simulink model "ElectroMechanics_Q_modified"  (R2024a)
settings: Solver=VariableStepAuto  StartTime=0.0  StopTime=40  RelTol=1e-3
libraries: fl_lib x15, nesl_utility x11, sdl_lib x4, ee_lib x4, batteryecm_lib x1, simulink x1
(part 2 of 2)

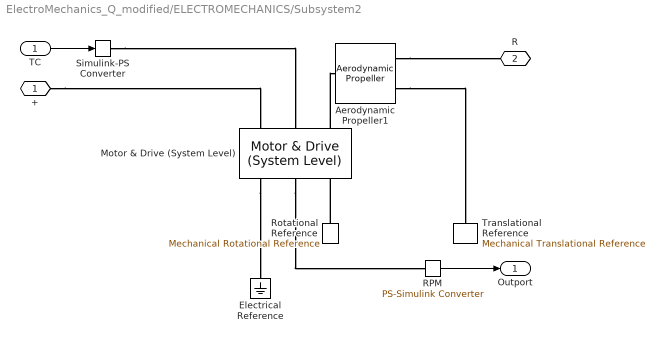
== system ElectroMechanics_Q_modified/ELECTROMECHANICS/Subsystem2 ==
  TC : Inport
  " Electrical Reference" : fl_lib/Electrical/Electrical Elements/Electrical Reference
  Aerodynamic Propeller1 : sdl_lib/Engines & Motors/Aerodynamic Propeller  parameterization=sdl.enum.AerodynamicPropellerParameterization.Constant  pitch_type=foundation.enum.constant_controlled.constant  direction=sdl.enum.PropellerDirection.Positive  root_pitch=0 deg  D=0.254 m  kt_const=0.110  kp_const=0.05655  kt_poly_fixed=[.002, .0006, -.0509, .0617]  kp_poly_fixed=[-.0752, .0577, -.0622, .16]  pitch_angle_TLU=[-15, 15, 25, 35, 45] deg  kt_poly_TLU=[.0002, -.00041, -.036, .03; .00026, -.00056, -.048, .04; .002, .00063, -.051, .062; .0014, -.0016, -.048, .087; .00087, -.0036, -.041, .12]  kp_poly_TLU=[-.1, .031, .0055, .088; -.081, -.025, .0044, .07; -.075, .058, -.062, .16; -.052, .065, -.08, .3; -.031, .057, -.069, .4]  J_TLU=[.01, .3, .625, 1.55, 2, 2.6]  kt_TLU_1D=[.0614, .0473, .0318, -.0127, -.0343, -.063]  kp_TLU_1D=[.1496, .1314, .116, -.0521, -.1503, -.2813]  kt_TLU_2D=[.00019, .013, .0048, -.017, -.03, -.045; .00039, .025, .0096, -.037, -.06, -.09; .00061, .047, .032, -.013, -.034, -.063; .00086, .072, .057, .014, -.0076, -.036; .12, .104, .09, .049, .029, .0019]  kp_TLU_2D=[.029, .029, .016, .06, .009, -.16; .059, .054, .031, -.12, -.19, -.29; .15, .13, .12, -.052, -.15, -.28; .26, .24, .22, .097, -.04, -.25; .39, .39, .38, .32, .24, .062]  beta_TLU=linspace(0, 360, 10) deg  Ct_TLU_1D=0.035 * sind(linspace(0, 360, 10) - 200)  Cq_TLU_1D=0.010 * sind(linspace(0, 360, 10) - 200)  Ct_TLU_2D=[0.01 * sind(linspace(0, 360, 10) - 200); 0.020 * sind(linspace(0, 360, 10) - 200); 0.035 * sind(linspace(0, 360, 10) - 200); 0.04 * sind(linspace(0, 360, 10) - 200); 0.06 * sind(linspace(0, 360, 10) - 200)]  Cq_TLU_2D=[0.0005 * sind(linspace(0, 360, 10) - 200); 0.0015 * sind(linspace(0, 360, 10) - 200); 0.0025 * sind(linspace(0, 360, 10) - 200); 0.0035 * sind(linspace(0, 360, 10) - 200); 0.0045 * sind(linspace(0, 360, 10) - 200)]  n_blades=2  n_blade_discretization=20  radial_TLU=[.1, .12, .2, .4, .6, .8, 1]  twist_TLU=[30, 35, 50, 30, 20, 15, 10] deg  chord_TLU=[.0676, .0666, .0824, .1025, .0885, .0598, .0133]  alpha_TLU=-180 : 10 : 180 deg  Cl_TLU=[.1326, .1326, .1274, .1274, .1274, .1274, .1274; .3626, .3626, .5002, .5002, .5002, .5002, .5002; .5528, .5528, .8007, .8007, .8007, .8007, .8007; .7256, .7256, 1.0125, 1.0125, 1.0125, 1.0125, 1.0125; .8016, .8016, 1.1556, 1.1556, 1.1556, 1.1556, 1.1556; .7873, .7873, 1.1604, 1.1604, 1.1604, 1.1604, 1.1604; .7031, .7031, 1.0493, 1.0493, 1.0493, 1.0493, 1.0493; .5423, .5423, .7973, .7973, .7973, .7973, .7973; .3537, .3537, .4332, .4332, .4332, .4332, .4332; .1155, .1155, -.0376, -.0376, -.0376, -.0376, -.0376; -.1045, -.1045, -.4096, -.4096, -.4096, -.4096, -.4096; -.2999, -.2999, -.672, -.672, -.672, -.672, -.672; -.4401, -.4401, -.9343, -.9343, -.9343, -.9343, -.9343; -.5186, -.5186, -1.0477, -1.0477, -1.0477, -1.0477, -1.0477; -.5303, -.5303, -1.0387, -1.0387, -1.0387, -1.0387, -1.0387; -.5073, -.5073, -.9565, -.9565, -.9565, -.9565, -.9565; -.442, -.442, -.7713, -.7713, -.7713, -.7713, -.7713; -.2658, -.2658, -.4832, -.4832, -.4832, -.4832, -.4832; .4109, .4109, .3629, .3629, .3629, .3629, .3629; 1.1635, 1.1635, 1.3779, 1.3779, 1.3779, 1.3779, 1.3779; 1.2412, 1.2412, 1.4033, 1.4033, 1.4033, 1.4033, 1.4033; .7434, .7434, 1.3453, 1.3453, 1.3453, 1.3453, 1.3453; .7908, .7908, 1.2862, 1.2862, 1.2862, 1.2862, 1.2862; .7525, .7525, 1.1562, 1.1562, 1.1562, 1.1562, 1.1562; .6722, .6722, .9487, .9487, .9487, .9487, .9487; .5324, .5324, .7047, .7047, .7047, .7047, .7047; .3365, .3365, .382, .382, .382, .382, .382; .0529, .0529, -.0229, -.0229, -.0229, -.0229, -.0229; -.2728, -.2728, -.316, -.316, -.316, -.316, -.316; -.4135, -.4135, -.6195, -.6195, -.6195, -.6195, -.6195; -.5087, -.5087, -.7847, -.7847, -.7847, -.7847, -.7847; -.5342, -.5342, -.8419, -.8419, -.8419, -.8419, -.8419; -.5166, -.5166, -.7658, -.7658, -.7658, -.7658, -.7658; -.4321, -.4321, -.5707, -.5707, -.5707, -.5707, -.5707; -.2864, -.2864, -.3098, -.3098, -.3098, -.3098, -.3098; -.1073, -.1073, -.0893, -.0893, -.0893, -.0893, -.0893; .1326, .1326, .1274, .1274, .1274, .1274, .1274]  Cd_TLU=[.0055, .0055, .3904, .3904, .3904, .3904, .3904; .0774, .0774, .449, .449, .449, .449, .449; .2412, .2412, .5915, .5915, .5915, .5915, .5915; .4342, .4342, .8307, .8307, .8307, .8307, .8307; .679, .679, 1.0909, 1.0909, 1.0909, 1.0909, 1.0909; .9003, .9003, 1.3868, 1.3868, 1.3868, 1.3868, 1.3868; 1.0825, 1.0825, 1.6565, 1.6565, 1.6565, 1.6565, 1.6565; 1.2281, 1.2281, 1.875, 1.875, 1.875, 1.875, 1.875; 1.3205, 1.3205, 2.017, 2.017, 2.017, 2.017, 2.017; 1.3234, 1.3234, 2.0407, 2.0407, 2.0407, 2.0407, 2.0407; 1.2391, 1.2391, 1.9513, 1.9513, 1.9513, 1.9513, 1.9513; 1.0963, 1.0963, 1.7643, 1.7643, 1.7643, 1.7643, 1.7643; .8978, .8978, 1.5048, 1.5048, 1.5048, 1.5048, 1.5048; .6525, .6525, 1.2281, 1.2281, 1.2281, 1.2281, 1.2281; .4203, .4203, .838, .838, .838, .838, .838; .2428, .2428, .5434, .5434, .5434, .5434, .5434; .0951, .0951, .2517, .2517, .2517, .2517, .2517; .0292, .0292, .0698, .0698, .0698, .0698, .0698; .0148, .0148, .0267, .0267, .0267, .0267, .0267; .0808, .0808, .0509, .0509, .0509, .0509, .0509; .2429, .2429, .1561, .1561, .1561, .1561, .1561; .5019, .5019, .3927, .3927, .3927, .3927, .3927; .7217, .7217, .7438, .7438, .7438, .7438, .7438; .9336, .9336, 1.1277, 1.1277, 1.1277, 1.1277, 1.1277; 1.0984, 1.0984, 1.4838, 1.4838, 1.4838, 1.4838, 1.4838; 1.2274, 1.2274, 1.7877, 1.7877, 1.7877, 1.7877, 1.7877; 1.3016, 1.3016, 1.9779, 1.9779, 1.9779, 1.9779, 1.9779; 1.3305, 1.3305, 2.0516, 2.0516, 2.0516, 2.0516, 2.0516; 1.2889, 1.2889, 1.9974, 1.9974, 1.9974, 1.9974, 1.9974; 1.1677, 1.1677, 1.8463, 1.8463, 1.8463, 1.8463, 1.8463; 1.0076, 1.0076, 1.5699, 1.5699, 1.5699, 1.5699, 1.5699; .8068, .8068, 1.2596, 1.2596, 1.2596, 1.2596, 1.2596; .5688, .5688, .9493, .9493, .9493, .9493, .9493; .3604, .3604, .6154, .6154, .6154, .6154, .6154; .1802, .1802, .5015, .5015, .5015, .5015, .5015; .0699, .0699, .4265, .4265, .4265, .4265, .4265; .0055, .0055, .3904, .3904, .3904, .3904, .3904]  interp_method=simscape.enum.interpolation.linear  extrap_method=simscape.enum.extrapolation.linear  density_spec=foundation.enum.constant_variable.constant  rho=1.225 kg/m^3  rotational_ports=sdl.enum.ConnectionType.Conserving  translational_ports=sdl.enum.ConnectionType.Conserving  model_inertia=true  propeller_inertia=0.00005 kg*m^2  propeller_mass=15 g  efficiency_sensor=false  n_thr=0.001 Hz  k_thr=0.001  P_thr=0.01 W  operation_check=simscape.enum.assert.action.warn  expose_port_C=false  w_specify=off  w_priority=None  w=0 rad/s  w_nominal_specify=off  w_nominal_value=1  w_nominal_unit=rad/s  Q_specify=off  Q_priority=None  Q=0 N*m  Q_nominal_specify=off  Q_nominal_value=1  Q_nominal_unit=N*m  v_specify=off  v_priority=None  v=0 m/s  v_nominal_specify=off  v_nominal_value=1  v_nominal_unit=m/s  thrust_specify=off  thrust_priority=None  thrust=0 N  thrust_nominal_specify=off  thrust_nominal_value=1  thrust_nominal_unit=N
      settings: InternalSimscapePortConfiguration="{\"Bottom\":[],\"Left\":[{\"id\":\"R1\",\"label\":\"R1\",\"type\":\"foundation.mechanical.rotational.rotational\"}],\"Right\":[{\"id\":\"R2\",\"label\":\"R2\",\"type\":\"foundation.mechanical.translational.translational\"},{\"id\":\"C2\",\"label\":\"C2\",\"type\":\"foundation.mechanical.translational.translational\"}],\"Top\":[]}"
  Motor & Drive (System Level) : ee_lib/Electromechanical/Motor & Drive (System Level)  torque_speed_param=ee.enum.electromech.envelope.torque_power  overtorque_param=ee.enum.electromech.overtorque.no  T_t=[.09, .08, .07, 0] N*m  T_t_intermittent=[.36, .32, .28, 0] N*m  T_t_2D=[.09, .09, .09; .08, .08, .08; .07, .07, .07; 0, 0, 0] N*m  T_t_intermittent_2D=[.36, .36, .36; .32, .32, .32; .28, .28, .28; 0, 0, 0] N*m  w_t=[0, 3750, 7500, 8000] rpm  vdc_t=[6, 12, 24] V  torque_max=0.5 N*m  power_max=450 W  torque_max_intermittent=0.4 N*m  power_max_intermittent=120 W  time_overtorque=30 s  time_recover=60 s  Tc=0.005 s  EnableSwitch=false  losses_param=1  eff=95  w_eff=6000 rpm  T_eff=116.5 mN*m  Piron=0 W  Pbase=0 W  w_eff_vec=[-8000, -4000, 0, 4000, 8000] rpm  T_eff_vec=[0, .03, .06, .09] N*m  v_eff_vec=[100, 250, 400] V  losses_mat=[1.49, 1.67, 2.21, 3.1; .42, .69, 1.14, 2.03; .06, .24, .78, 1.68; .42, .69, 1.14, 2.03; 1.49, 1.67, 2.21, 3.1] W  efficiency_mat=[95, 95, 95, 95; 95, 95, 95, 95; 95, 95, 95, 95; 95, 95, 95, 95; 95, 95, 95, 95]  losses_mat_3D=ones(5, 4, 3) W  efficiency_mat_3D=95 * ones(5, 4, 3)  Res=0.085 Ohm  enable_fault=simscape.enum.onoff.off  fault_condition=1  fault_threshold=0.5  J=1.5e-5 kg*m^2  lam=2.5e-8 N*m*s/rad  speed0=0 rpm  faulted_specify=off  faulted_priority=None  faulted=0  faulted_nominal_specify=off  faulted_nominal_value=1  faulted_nominal_unit=1  isSwitchedOff_specify=off  isSwitchedOff_priority=None  isSwitchedOff=0  isSwitchedOff_nominal_specify=off  isSwitchedOff_nominal_value=1  isSwitchedOff_nominal_unit=1  torqueLimitContinuous_specify=off  torqueLimitContinuous_priority=None  torqueLimitContinuous=0 N*m  torqueLimitContinuous_nominal_specify=off  torqueLimitContinuous_nominal_value=1  torqueLimitContinuous_nominal_unit=N*m  alpha=3.93e-3 1/K  Tmeas=25 degC  Tmeas2=125 degC  losses_mat_T2=[1.49, 1.74, 2.49, 3.74; .42, .67, 1.42, 2.67; .06, .31, 1.06, 2.31; .42, .67, 1.42, 2.67; 1.49, 1.74, 2.49, 3.74] W  efficiency_mat_T2=[95, 95, 95, 95; 95, 95, 95, 95; 95, 95, 95, 95; 95, 95, 95, 95; 95, 95, 95, 95]  losses_mat_3D_T2=ones(5, 4, 3) W  efficiency_mat_3D_T2=95 * ones(5, 4, 3)  thermal_mass=100 J/K  initial_temperature=25 degC
  RPM : nesl_utility/PS-Simulink Converter  PhysicalDomain=network_engine_domain  SubClassName=ps_output  LeftPortType=input  RightPortType=output  PseudoPeriodic=off  Frequencies=[]  VectorFormat=inherit  Unit=rpm  AffineConversion=off
  Rotational Reference : fl_lib/Mechanical/Rotational Elements/Mechanical Rotational Reference
  Simulink-PS Converter : nesl_utility/Simulink-PS Converter  PhysicalDomain=network_engine_domain  SubClassName=ps_input  LeftPortType=input  RightPortType=output  PseudoPeriodic=off  Frequencies=[]  NoiseDistribution=none  NoiseParameters=[]  Unit=1  AffineConversion=off  FilteringAndDerivatives=provide  SimscapeFilterOrder=1  InputFilterTimeConstant=0.001  UdotUserProvided=0
  Translational Reference : fl_lib/Mechanical/Translational Elements/Mechanical Translational Reference
  + : PMIOPort  Side=Left
  R : PMIOPort  Port=2  Side=Right
  Outport : Outport
  wires:
  RPM/1 -> Outport/1
  TC/1 -> Simulink-PS Converter/1
  connections:
  Aerodynamic Propeller1/RConn2 -- Translational Reference/LConn1
  Rotational Reference/LConn1 -- Motor & Drive (System Level)/RConn3
  Motor & Drive (System Level)/RConn1 -- " Electrical Reference"/LConn1
  Motor & Drive (System Level)/LConn3 -- Aerodynamic Propeller1/LConn1
  Motor & Drive (System Level)/RConn2 -- RPM/LConn1
  +/RConn1 -- Motor & Drive (System Level)/LConn1
  Aerodynamic Propeller1/RConn1 -- R/RConn1
  Simulink-PS Converter/RConn1 -- Motor & Drive (System Level)/LConn2

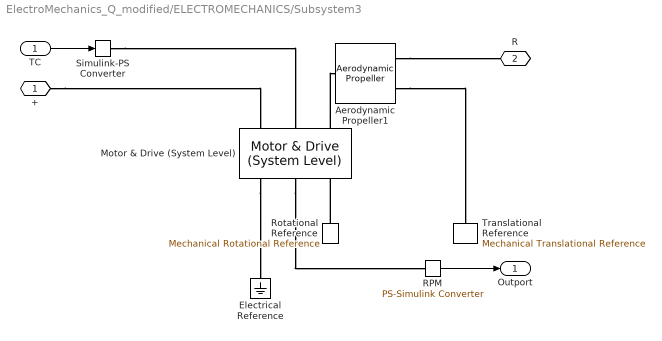
== system ElectroMechanics_Q_modified/ELECTROMECHANICS/Subsystem3 ==
  TC : Inport
  " Electrical Reference" : fl_lib/Electrical/Electrical Elements/Electrical Reference
  Aerodynamic Propeller1 : sdl_lib/Engines & Motors/Aerodynamic Propeller  parameterization=sdl.enum.AerodynamicPropellerParameterization.Constant  pitch_type=foundation.enum.constant_controlled.constant  direction=sdl.enum.PropellerDirection.Positive  root_pitch=0 deg  D=0.254 m  kt_const=0.110  kp_const=0.05655  kt_poly_fixed=[.002, .0006, -.0509, .0617]  kp_poly_fixed=[-.0752, .0577, -.0622, .16]  pitch_angle_TLU=[-15, 15, 25, 35, 45] deg  kt_poly_TLU=[.0002, -.00041, -.036, .03; .00026, -.00056, -.048, .04; .002, .00063, -.051, .062; .0014, -.0016, -.048, .087; .00087, -.0036, -.041, .12]  kp_poly_TLU=[-.1, .031, .0055, .088; -.081, -.025, .0044, .07; -.075, .058, -.062, .16; -.052, .065, -.08, .3; -.031, .057, -.069, .4]  J_TLU=[.01, .3, .625, 1.55, 2, 2.6]  kt_TLU_1D=[.0614, .0473, .0318, -.0127, -.0343, -.063]  kp_TLU_1D=[.1496, .1314, .116, -.0521, -.1503, -.2813]  kt_TLU_2D=[.00019, .013, .0048, -.017, -.03, -.045; .00039, .025, .0096, -.037, -.06, -.09; .00061, .047, .032, -.013, -.034, -.063; .00086, .072, .057, .014, -.0076, -.036; .12, .104, .09, .049, .029, .0019]  kp_TLU_2D=[.029, .029, .016, .06, .009, -.16; .059, .054, .031, -.12, -.19, -.29; .15, .13, .12, -.052, -.15, -.28; .26, .24, .22, .097, -.04, -.25; .39, .39, .38, .32, .24, .062]  beta_TLU=linspace(0, 360, 10) deg  Ct_TLU_1D=0.035 * sind(linspace(0, 360, 10) - 200)  Cq_TLU_1D=0.010 * sind(linspace(0, 360, 10) - 200)  Ct_TLU_2D=[0.01 * sind(linspace(0, 360, 10) - 200); 0.020 * sind(linspace(0, 360, 10) - 200); 0.035 * sind(linspace(0, 360, 10) - 200); 0.04 * sind(linspace(0, 360, 10) - 200); 0.06 * sind(linspace(0, 360, 10) - 200)]  Cq_TLU_2D=[0.0005 * sind(linspace(0, 360, 10) - 200); 0.0015 * sind(linspace(0, 360, 10) - 200); 0.0025 * sind(linspace(0, 360, 10) - 200); 0.0035 * sind(linspace(0, 360, 10) - 200); 0.0045 * sind(linspace(0, 360, 10) - 200)]  n_blades=2  n_blade_discretization=20  radial_TLU=[.1, .12, .2, .4, .6, .8, 1]  twist_TLU=[30, 35, 50, 30, 20, 15, 10] deg  chord_TLU=[.0676, .0666, .0824, .1025, .0885, .0598, .0133]  alpha_TLU=-180 : 10 : 180 deg  Cl_TLU=[.1326, .1326, .1274, .1274, .1274, .1274, .1274; .3626, .3626, .5002, .5002, .5002, .5002, .5002; .5528, .5528, .8007, .8007, .8007, .8007, .8007; .7256, .7256, 1.0125, 1.0125, 1.0125, 1.0125, 1.0125; .8016, .8016, 1.1556, 1.1556, 1.1556, 1.1556, 1.1556; .7873, .7873, 1.1604, 1.1604, 1.1604, 1.1604, 1.1604; .7031, .7031, 1.0493, 1.0493, 1.0493, 1.0493, 1.0493; .5423, .5423, .7973, .7973, .7973, .7973, .7973; .3537, .3537, .4332, .4332, .4332, .4332, .4332; .1155, .1155, -.0376, -.0376, -.0376, -.0376, -.0376; -.1045, -.1045, -.4096, -.4096, -.4096, -.4096, -.4096; -.2999, -.2999, -.672, -.672, -.672, -.672, -.672; -.4401, -.4401, -.9343, -.9343, -.9343, -.9343, -.9343; -.5186, -.5186, -1.0477, -1.0477, -1.0477, -1.0477, -1.0477; -.5303, -.5303, -1.0387, -1.0387, -1.0387, -1.0387, -1.0387; -.5073, -.5073, -.9565, -.9565, -.9565, -.9565, -.9565; -.442, -.442, -.7713, -.7713, -.7713, -.7713, -.7713; -.2658, -.2658, -.4832, -.4832, -.4832, -.4832, -.4832; .4109, .4109, .3629, .3629, .3629, .3629, .3629; 1.1635, 1.1635, 1.3779, 1.3779, 1.3779, 1.3779, 1.3779; 1.2412, 1.2412, 1.4033, 1.4033, 1.4033, 1.4033, 1.4033; .7434, .7434, 1.3453, 1.3453, 1.3453, 1.3453, 1.3453; .7908, .7908, 1.2862, 1.2862, 1.2862, 1.2862, 1.2862; .7525, .7525, 1.1562, 1.1562, 1.1562, 1.1562, 1.1562; .6722, .6722, .9487, .9487, .9487, .9487, .9487; .5324, .5324, .7047, .7047, .7047, .7047, .7047; .3365, .3365, .382, .382, .382, .382, .382; .0529, .0529, -.0229, -.0229, -.0229, -.0229, -.0229; -.2728, -.2728, -.316, -.316, -.316, -.316, -.316; -.4135, -.4135, -.6195, -.6195, -.6195, -.6195, -.6195; -.5087, -.5087, -.7847, -.7847, -.7847, -.7847, -.7847; -.5342, -.5342, -.8419, -.8419, -.8419, -.8419, -.8419; -.5166, -.5166, -.7658, -.7658, -.7658, -.7658, -.7658; -.4321, -.4321, -.5707, -.5707, -.5707, -.5707, -.5707; -.2864, -.2864, -.3098, -.3098, -.3098, -.3098, -.3098; -.1073, -.1073, -.0893, -.0893, -.0893, -.0893, -.0893; .1326, .1326, .1274, .1274, .1274, .1274, .1274]  Cd_TLU=[.0055, .0055, .3904, .3904, .3904, .3904, .3904; .0774, .0774, .449, .449, .449, .449, .449; .2412, .2412, .5915, .5915, .5915, .5915, .5915; .4342, .4342, .8307, .8307, .8307, .8307, .8307; .679, .679, 1.0909, 1.0909, 1.0909, 1.0909, 1.0909; .9003, .9003, 1.3868, 1.3868, 1.3868, 1.3868, 1.3868; 1.0825, 1.0825, 1.6565, 1.6565, 1.6565, 1.6565, 1.6565; 1.2281, 1.2281, 1.875, 1.875, 1.875, 1.875, 1.875; 1.3205, 1.3205, 2.017, 2.017, 2.017, 2.017, 2.017; 1.3234, 1.3234, 2.0407, 2.0407, 2.0407, 2.0407, 2.0407; 1.2391, 1.2391, 1.9513, 1.9513, 1.9513, 1.9513, 1.9513; 1.0963, 1.0963, 1.7643, 1.7643, 1.7643, 1.7643, 1.7643; .8978, .8978, 1.5048, 1.5048, 1.5048, 1.5048, 1.5048; .6525, .6525, 1.2281, 1.2281, 1.2281, 1.2281, 1.2281; .4203, .4203, .838, .838, .838, .838, .838; .2428, .2428, .5434, .5434, .5434, .5434, .5434; .0951, .0951, .2517, .2517, .2517, .2517, .2517; .0292, .0292, .0698, .0698, .0698, .0698, .0698; .0148, .0148, .0267, .0267, .0267, .0267, .0267; .0808, .0808, .0509, .0509, .0509, .0509, .0509; .2429, .2429, .1561, .1561, .1561, .1561, .1561; .5019, .5019, .3927, .3927, .3927, .3927, .3927; .7217, .7217, .7438, .7438, .7438, .7438, .7438; .9336, .9336, 1.1277, 1.1277, 1.1277, 1.1277, 1.1277; 1.0984, 1.0984, 1.4838, 1.4838, 1.4838, 1.4838, 1.4838; 1.2274, 1.2274, 1.7877, 1.7877, 1.7877, 1.7877, 1.7877; 1.3016, 1.3016, 1.9779, 1.9779, 1.9779, 1.9779, 1.9779; 1.3305, 1.3305, 2.0516, 2.0516, 2.0516, 2.0516, 2.0516; 1.2889, 1.2889, 1.9974, 1.9974, 1.9974, 1.9974, 1.9974; 1.1677, 1.1677, 1.8463, 1.8463, 1.8463, 1.8463, 1.8463; 1.0076, 1.0076, 1.5699, 1.5699, 1.5699, 1.5699, 1.5699; .8068, .8068, 1.2596, 1.2596, 1.2596, 1.2596, 1.2596; .5688, .5688, .9493, .9493, .9493, .9493, .9493; .3604, .3604, .6154, .6154, .6154, .6154, .6154; .1802, .1802, .5015, .5015, .5015, .5015, .5015; .0699, .0699, .4265, .4265, .4265, .4265, .4265; .0055, .0055, .3904, .3904, .3904, .3904, .3904]  interp_method=simscape.enum.interpolation.linear  extrap_method=simscape.enum.extrapolation.linear  density_spec=foundation.enum.constant_variable.constant  rho=1.225 kg/m^3  rotational_ports=sdl.enum.ConnectionType.Conserving  translational_ports=sdl.enum.ConnectionType.Conserving  model_inertia=true  propeller_inertia=0.00005 kg*m^2  propeller_mass=15 g  efficiency_sensor=false  n_thr=0.001 Hz  k_thr=0.001  P_thr=0.01 W  operation_check=simscape.enum.assert.action.warn  expose_port_C=false  w_specify=off  w_priority=None  w=0 rad/s  w_nominal_specify=off  w_nominal_value=1  w_nominal_unit=rad/s  Q_specify=off  Q_priority=None  Q=0 N*m  Q_nominal_specify=off  Q_nominal_value=1  Q_nominal_unit=N*m  v_specify=off  v_priority=None  v=0 m/s  v_nominal_specify=off  v_nominal_value=1  v_nominal_unit=m/s  thrust_specify=off  thrust_priority=None  thrust=0 N  thrust_nominal_specify=off  thrust_nominal_value=1  thrust_nominal_unit=N
      settings: InternalSimscapePortConfiguration="{\"Bottom\":[],\"Left\":[{\"id\":\"R1\",\"label\":\"R1\",\"type\":\"foundation.mechanical.rotational.rotational\"}],\"Right\":[{\"id\":\"R2\",\"label\":\"R2\",\"type\":\"foundation.mechanical.translational.translational\"},{\"id\":\"C2\",\"label\":\"C2\",\"type\":\"foundation.mechanical.translational.translational\"}],\"Top\":[]}"
  Motor & Drive (System Level) : ee_lib/Electromechanical/Motor & Drive (System Level)  torque_speed_param=ee.enum.electromech.envelope.torque_power  overtorque_param=ee.enum.electromech.overtorque.no  T_t=[.09, .08, .07, 0] N*m  T_t_intermittent=[.36, .32, .28, 0] N*m  T_t_2D=[.09, .09, .09; .08, .08, .08; .07, .07, .07; 0, 0, 0] N*m  T_t_intermittent_2D=[.36, .36, .36; .32, .32, .32; .28, .28, .28; 0, 0, 0] N*m  w_t=[0, 3750, 7500, 8000] rpm  vdc_t=[6, 12, 24] V  torque_max=0.5 N*m  power_max=450 W  torque_max_intermittent=0.4 N*m  power_max_intermittent=120 W  time_overtorque=30 s  time_recover=60 s  Tc=0.005 s  EnableSwitch=false  losses_param=1  eff=95  w_eff=6000 rpm  T_eff=116.5 mN*m  Piron=0 W  Pbase=0 W  w_eff_vec=[-8000, -4000, 0, 4000, 8000] rpm  T_eff_vec=[0, .03, .06, .09] N*m  v_eff_vec=[100, 250, 400] V  losses_mat=[1.49, 1.67, 2.21, 3.1; .42, .69, 1.14, 2.03; .06, .24, .78, 1.68; .42, .69, 1.14, 2.03; 1.49, 1.67, 2.21, 3.1] W  efficiency_mat=[95, 95, 95, 95; 95, 95, 95, 95; 95, 95, 95, 95; 95, 95, 95, 95; 95, 95, 95, 95]  losses_mat_3D=ones(5, 4, 3) W  efficiency_mat_3D=95 * ones(5, 4, 3)  Res=0.085 Ohm  enable_fault=simscape.enum.onoff.off  fault_condition=1  fault_threshold=0.5  J=1.5e-5 kg*m^2  lam=2.5e-8 N*m*s/rad  speed0=0 rpm  faulted_specify=off  faulted_priority=None  faulted=0  faulted_nominal_specify=off  faulted_nominal_value=1  faulted_nominal_unit=1  isSwitchedOff_specify=off  isSwitchedOff_priority=None  isSwitchedOff=0  isSwitchedOff_nominal_specify=off  isSwitchedOff_nominal_value=1  isSwitchedOff_nominal_unit=1  torqueLimitContinuous_specify=off  torqueLimitContinuous_priority=None  torqueLimitContinuous=0 N*m  torqueLimitContinuous_nominal_specify=off  torqueLimitContinuous_nominal_value=1  torqueLimitContinuous_nominal_unit=N*m  alpha=3.93e-3 1/K  Tmeas=25 degC  Tmeas2=125 degC  losses_mat_T2=[1.49, 1.74, 2.49, 3.74; .42, .67, 1.42, 2.67; .06, .31, 1.06, 2.31; .42, .67, 1.42, 2.67; 1.49, 1.74, 2.49, 3.74] W  efficiency_mat_T2=[95, 95, 95, 95; 95, 95, 95, 95; 95, 95, 95, 95; 95, 95, 95, 95; 95, 95, 95, 95]  losses_mat_3D_T2=ones(5, 4, 3) W  efficiency_mat_3D_T2=95 * ones(5, 4, 3)  thermal_mass=100 J/K  initial_temperature=25 degC
  RPM : nesl_utility/PS-Simulink Converter  PhysicalDomain=network_engine_domain  SubClassName=ps_output  LeftPortType=input  RightPortType=output  PseudoPeriodic=off  Frequencies=[]  VectorFormat=inherit  Unit=rpm  AffineConversion=off
  Rotational Reference : fl_lib/Mechanical/Rotational Elements/Mechanical Rotational Reference
  Simulink-PS Converter : nesl_utility/Simulink-PS Converter  PhysicalDomain=network_engine_domain  SubClassName=ps_input  LeftPortType=input  RightPortType=output  PseudoPeriodic=off  Frequencies=[]  NoiseDistribution=none  NoiseParameters=[]  Unit=1  AffineConversion=off  FilteringAndDerivatives=provide  SimscapeFilterOrder=1  InputFilterTimeConstant=0.001  UdotUserProvided=0
  Translational Reference : fl_lib/Mechanical/Translational Elements/Mechanical Translational Reference
  + : PMIOPort  Side=Left
  R : PMIOPort  Port=2  Side=Right
  Outport : Outport
  wires:
  RPM/1 -> Outport/1
  TC/1 -> Simulink-PS Converter/1
  connections:
  Aerodynamic Propeller1/RConn2 -- Translational Reference/LConn1
  Rotational Reference/LConn1 -- Motor & Drive (System Level)/RConn3
  Motor & Drive (System Level)/RConn1 -- " Electrical Reference"/LConn1
  Motor & Drive (System Level)/LConn3 -- Aerodynamic Propeller1/LConn1
  Motor & Drive (System Level)/RConn2 -- RPM/LConn1
  +/RConn1 -- Motor & Drive (System Level)/LConn1
  Aerodynamic Propeller1/RConn1 -- R/RConn1
  Simulink-PS Converter/RConn1 -- Motor & Drive (System Level)/LConn2
